simulink model "single_phase_afe_ideal"  (R2026a)
settings: Solver=ode23tb  StopTime=simlength  FixedStep=tc  MaxStep=glb_time.tc
values from neighbouring files (symbols this model uses):
  afe_ctrl = ctrl_afe_setup(glb_time.ts_afe, grid_emu.omega_grid_nom)    [init_model_legacy.m]
  frequency_set = 300    [init_model_legacy.m]
  glb_time = timing_setup(fpwm_afe, trgo_afe, fpwm_inv, trgo_inv, fpwm_single_phase_inv, trgo_single_phase_inv, fpwm_dab, trgo_dab,      fpwm_psfbc, trgo_psfbc, fpwm_isop_rail, trgo_isop_rail, fpwm_cllc, trgo_cllc, t_measure, tc_factor, tc_decimation, delay_pwm, dead_time_afe,      dead_time_inv, dead_time_single_phase_inv, dead_time_dab, dead_time_psfbc, dead_time_isop_rail, dead_time_cllc)    [init_model_legacy.m]
  grid_emu = grid_three_phase_emulator('Dyn11', delta_star, grid_nominal_power, application_voltage, us1, us2, fgrid,                  eq_grid_inductance, eq_grid_resistance, eta, ucc, i1m, p_iron, n1, n2, core_area, core_length, mur,                  up_xi_pu_ref, up_eta_pu_ref, un_xi_pu_ref, un_eta_pu_ref)    [init_model_legacy.m]
  heatsink = liquid_cooled_plate_2kw_setup(weight, no_weight, cp_al, heat_capacity_hs, thermal_conductivity_al,      Rth_switch_HA, Rth_mosfet_HA, Rth_diode_HA, Tambient, DThs_init)    [init_model_legacy.m]
  kepsilon = 2    [init_model_legacy.m]
  omega_set = frequency_set*2*pi    (= 1884.95559215)    [init_model_legacy.m]
  single_phase_inverter_ctrl = ctrl_single_phase_inverter_setup(glb_time.ts_inv, pres_ctrl.omega_set,      dqvector_pi.kp_inv, dqvector_pi.ki_inv, pres_ctrl.kp_rpi, pres_ctrl.ki_rpi, pres_ctrl.delta_rpi)    [init_model_legacy.m]
  Tambient = 40    [init_model_legacy.m]
  time_step_ref_1 = 0.025    [init_model_legacy.m]
  time_step_ref_2 = 0.5    [init_model_legacy.m]
  time_step_ref_3 = 1    [init_model_legacy.m]
  Vdc_nom = 400*1.35    (= 540)    [power_losses_calculation.m]
undefined symbols (not defined in the file or in its folder): delta_fht1, hwdata, igbt, Ld_fht1, magnitude, omega_fht1, ts_inv, Vac_FS, Xbez
libraries: fl_lib x116, nesl_utility x65, phase_shift_filter_ccaller x5, dq_vector_pi x4, igbt_simple_2th_lib x4, linear_double_integrator_observer_ccaller x3, lithium_ion_battery x1, dclink_for_two_levels x1, three_phase_voltage_with_frt_emulator x1, simulink x1, cstblocks_lti x1, single_phase_pwm_modulator x1
(part 5 of 6)

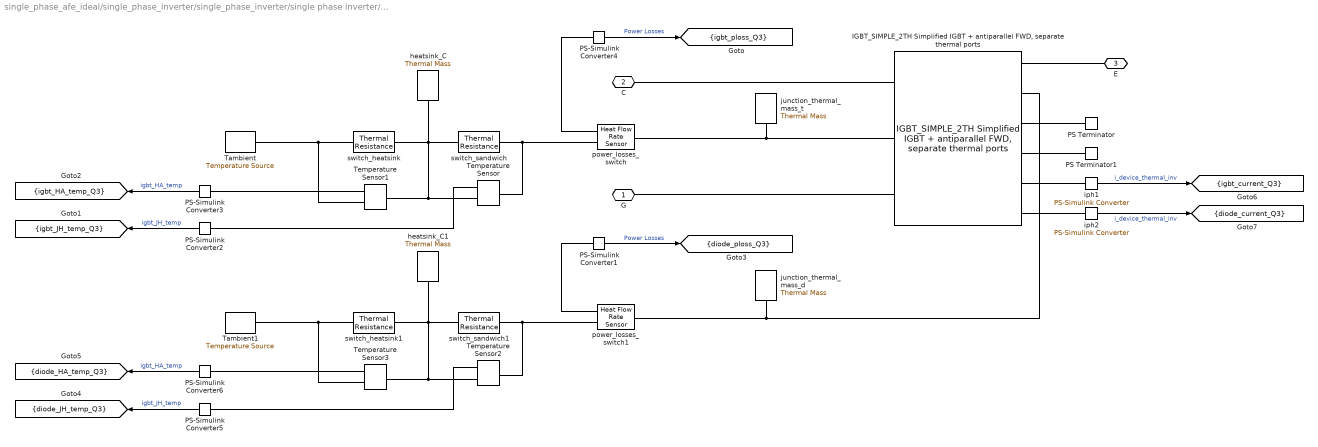
== system single_phase_afe_ideal/single_phase_inverter/single_phase_inverter/single phase inverter/three_phase_inverter_with_igbt_simple_2th/full_bridge_with_igbt_simple_2th/igbt_simple_3/IGBT_simple ==
  "IGBT_SIMPLE_2TH Simplified IGBT + antiparallel FWD, separate thermal ports" : igbt_simple_2th_lib/IGBT_SIMPLE_2TH Simplified IGBT + antiparallel FWD, separate thermal ports  Vce_sat=vce_sat_m V  Vf=v_gamma_m V  Vth=Vth_gate_m V  Vhyst=Vth_gate_hyst_m V  Eon_ref=Eon_m mJ  Eoff_ref=Eoff_m mJ  Err_ref=Err_m mJ  Ic_ref=Ic_ref_m A  Vdc_ref=Vdc_ref_m V  V_rr_th=Vblock_Errf_m V  Ron=rce_on_m mOhm  Rd=rd_on_m mOhm  Goff=Gce_off_m 1/Ohm  tau_s=time_constant_edge_m us  tau_p=time_constant_ploss_m us  i_specify=off  i_priority=None  i=0 A  i_nominal_specify=off  i_nominal_value=1  i_nominal_unit=A  v_specify=off  v_priority=None  v=0 V  v_nominal_specify=off  v_nominal_value=1  v_nominal_unit=V  i_t_specify=off  i_t_priority=None  i_t=0 A  i_t_nominal_specify=off  i_t_nominal_value=1  i_t_nominal_unit=A  i_d_specify=off  i_d_priority=None  i_d=0 A  i_d_nominal_specify=off  i_d_nominal_value=1  i_d_nominal_unit=A  i_h_specify=off  i_h_priority=None  i_h=0 A  i_h_nominal_specify=off  i_h_nominal_value=1  i_h_nominal_unit=A  i_dh_specify=off  i_dh_priority=None  i_dh=0 A  i_dh_nominal_specify=off  i_dh_nominal_value=1  i_dh_nominal_unit=A  v_h_specify=off  v_h_priority=None  v_h=0 V  v_h_nominal_specify=off  v_h_nominal_value=1  v_h_nominal_unit=V  E_lpt_specify=off  E_lpt_priority=None  E_lpt=0 J  E_lpt_nominal_specify=off  E_lpt_nominal_value=1  E_lpt_nominal_unit=J  E_lpd_specify=off  E_lpd_priority=None  E_lpd=0 J  E_lpd_nominal_specify=off  E_lpd_nominal_value=1  E_lpd_nominal_unit=J  Qt_specify=off  Qt_priority=None  Qt=0 W  Qt_nominal_specify=off  Qt_nominal_value=1  Qt_nominal_unit=W  Qd_specify=off  Qd_priority=None  Qd=0 W  Qd_nominal_specify=off  Qd_nominal_value=1  Qd_nominal_unit=W  E_t_specify=off  E_t_priority=None  E_t=0 J  E_d_specify=off  E_d_priority=None  E_d=0 J
  PS Terminator : fl_lib/Physical Signals/Sinks/PS Terminator
  PS Terminator1 : fl_lib/Physical Signals/Sinks/PS Terminator
  PS-Simulink Converter1 : nesl_utility/PS-Simulink Converter  PhysicalDomain=network_engine_domain  SubClassName=ps_output  LeftPortType=input  RightPortType=output  PseudoPeriodic=off  Frequencies=[]  VectorFormat=1-D array  Unit=J/s  AffineConversion=off
  PS-Simulink Converter{2..3,5..6} (4 alike) : nesl_utility/PS-Simulink Converter  PhysicalDomain=network_engine_domain  SubClassName=ps_output  LeftPortType=input  RightPortType=output  PseudoPeriodic=off  Frequencies=[]  VectorFormat=1-D array  Unit=degC  AffineConversion=off
  PS-Simulink Converter4 : nesl_utility/PS-Simulink Converter  PhysicalDomain=network_engine_domain  SubClassName=ps_output  LeftPortType=input  RightPortType=output  PseudoPeriodic=off  Frequencies=[]  VectorFormat=1-D array  Unit=J/s  AffineConversion=off
  Tambient : fl_lib/Thermal/Thermal Sources/Temperature Source  temperature=Tambient_m degC
  Tambient1 : fl_lib/Thermal/Thermal Sources/Temperature Source  temperature=Tambient_m degC
  Temperature Sensor{,1..3} (4 alike) : fl_lib/Thermal/Thermal Sensors/Temperature Sensor  temperature_measure=foundation.enum.MeasurementReference.difference
  heatsink_C : fl_lib/Thermal/Thermal Elements/Thermal Mass  mass_type=foundation.enum.constant_variable.constant  mass=mass_heatsink_m kg  sp_heat=specific_heat_m J/(K*kg)  mass_min=1e-6 kg  num_ports=foundation.enum.numPorts2.one  m_specify=off  m_priority=High  m=1 kg  m_nominal_specify=off  m_nominal_value=1  m_nominal_unit=kg  T_specify=on  T_priority=High  T=Tambient_m degC  T_nominal_specify=off  T_nominal_value=1  T_nominal_unit=K  Q_specify=off  Q_priority=High  Q=0 W  Q_nominal_specify=off  Q_nominal_value=1  Q_nominal_unit=W
  heatsink_C1 : fl_lib/Thermal/Thermal Elements/Thermal Mass  mass_type=foundation.enum.constant_variable.constant  mass=mass_heatsink_m kg  sp_heat=specific_heat_m J/(K*kg)  mass_min=1e-6 kg  num_ports=foundation.enum.numPorts2.one  m_specify=off  m_priority=High  m=1 kg  m_nominal_specify=off  m_nominal_value=1  m_nominal_unit=kg  T_specify=on  T_priority=High  T=Tambient_m degC  T_nominal_specify=off  T_nominal_value=1  T_nominal_unit=K  Q_specify=off  Q_priority=High  Q=0 W  Q_nominal_specify=off  Q_nominal_value=1  Q_nominal_unit=W
  iph1 : nesl_utility/PS-Simulink Converter  PhysicalDomain=network_engine_domain  SubClassName=ps_output  LeftPortType=input  RightPortType=output  PseudoPeriodic=off  Frequencies=[]  VectorFormat=1-D array  Unit=A  AffineConversion=off
  iph2 : nesl_utility/PS-Simulink Converter  PhysicalDomain=network_engine_domain  SubClassName=ps_output  LeftPortType=input  RightPortType=output  PseudoPeriodic=off  Frequencies=[]  VectorFormat=1-D array  Unit=A  AffineConversion=off
  junction_thermal_mass_d : fl_lib/Thermal/Thermal Elements/Thermal Mass  mass_type=foundation.enum.constant_variable.constant  mass=JunctionTermalMass_m/specific_heat_m kg  sp_heat=specific_heat_m J/(K*kg)  mass_min=1e-6 kg  num_ports=foundation.enum.numPorts2.one  m_specify=off  m_priority=High  m=1 kg  m_nominal_specify=off  m_nominal_value=1  m_nominal_unit=kg  T_specify=on  T_priority=High  T=Tambient_m degC  T_nominal_specify=off  T_nominal_value=1  T_nominal_unit=K  Q_specify=off  Q_priority=High  Q=0 W  Q_nominal_specify=off  Q_nominal_value=1  Q_nominal_unit=W
  junction_thermal_mass_t : fl_lib/Thermal/Thermal Elements/Thermal Mass  mass_type=foundation.enum.constant_variable.constant  mass=JunctionTermalMass_m/specific_heat_m kg  sp_heat=specific_heat_m J/(K*kg)  mass_min=1e-6 kg  num_ports=foundation.enum.numPorts2.one  m_specify=off  m_priority=High  m=1 kg  m_nominal_specify=off  m_nominal_value=1  m_nominal_unit=kg  T_specify=on  T_priority=High  T=Tambient_m degC  T_nominal_specify=off  T_nominal_value=1  T_nominal_unit=K  Q_specify=off  Q_priority=High  Q=0 W  Q_nominal_specify=off  Q_nominal_value=1  Q_nominal_unit=W
  power_losses_switch : fl_lib/Thermal/Thermal Sensors/Heat Flow Rate Sensor
  power_losses_switch1 : fl_lib/Thermal/Thermal Sensors/Heat Flow Rate Sensor
  switch_heatsink : fl_lib/Thermal/Thermal Elements/Thermal Resistance  resistance=rth_switch_HA_m K/W  T_specify=off  T_priority=High  T=0 deltadegC  T_nominal_specify=off  T_nominal_value=1  T_nominal_unit=K  Q_specify=off  Q_priority=None  Q=0 W  Q_nominal_specify=off  Q_nominal_value=1  Q_nominal_unit=W
  switch_heatsink1 : fl_lib/Thermal/Thermal Elements/Thermal Resistance  resistance=rth_diode_HA_m K/W  T_specify=off  T_priority=High  T=0 deltadegC  T_nominal_specify=off  T_nominal_value=1  T_nominal_unit=K  Q_specify=off  Q_priority=None  Q=0 W  Q_nominal_specify=off  Q_nominal_value=1  Q_nominal_unit=W
  switch_sandwich : fl_lib/Thermal/Thermal Elements/Thermal Resistance  resistance=rth_switch_JH_m K/W  T_specify=off  T_priority=High  T=0 degC  T_nominal_specify=off  T_nominal_value=1  T_nominal_unit=K  Q_specify=off  Q_priority=None  Q=0 W  Q_nominal_specify=off  Q_nominal_value=1  Q_nominal_unit=W
  switch_sandwich1 : fl_lib/Thermal/Thermal Elements/Thermal Resistance  resistance=rth_diode_JH_m K/W  T_specify=off  T_priority=High  T=0 degC  T_nominal_specify=off  T_nominal_value=1  T_nominal_unit=K  Q_specify=off  Q_priority=None  Q=0 W  Q_nominal_specify=off  Q_nominal_value=1  Q_nominal_unit=W
  G : PMIOPort  Side=Left
  C : PMIOPort  Port=2  Side=Left
  E : PMIOPort  Port=3  Side=Right
  tag scope: diode_HA_temp_Q3=scoped, diode_JH_temp_Q3=scoped, diode_current_Q3=scoped, diode_ploss_Q3=scoped, igbt_HA_temp_Q3=scoped, igbt_JH_temp_Q3=scoped, igbt_current_Q3=scoped, igbt_ploss_Q3=scoped
  wires:
  PS-Simulink Converter3/1 -> [igbt_HA_temp_Q3]  "igbt_HA_temp"
  PS-Simulink Converter4/1 -> [igbt_ploss_Q3]  "Power Losses"
  PS-Simulink Converter2/1 -> [igbt_JH_temp_Q3]  "igbt_JH_temp"
  PS-Simulink Converter1/1 -> [diode_ploss_Q3]  "Power Losses"
  PS-Simulink Converter5/1 -> [diode_JH_temp_Q3]  "igbt_JH_temp"
  PS-Simulink Converter6/1 -> [diode_HA_temp_Q3]  "igbt_HA_temp"
  iph1/1 -> [igbt_current_Q3]  "i_device_thermal_inv"
  iph2/1 -> [diode_current_Q3]  "i_device_thermal_inv"
  connections:
  Temperature Sensor/RConn2 -- PS-Simulink Converter2/LConn1
  "IGBT_SIMPLE_2TH Simplified IGBT + antiparallel FWD, separate thermal ports"/LConn2 -- junction_thermal_mass_t/LConn1 -- power_losses_switch/LConn1
  Temperature Sensor1/RConn2 -- PS-Simulink Converter3/LConn1
  switch_heatsink/LConn1 -- heatsink_C/LConn1 -- switch_sandwich/RConn1 -- Temperature Sensor1/LConn1 -- Temperature Sensor/RConn1
  switch_heatsink/RConn1 -- Tambient/LConn1 -- Temperature Sensor1/RConn1
  switch_sandwich/LConn1 -- power_losses_switch/RConn2 -- Temperature Sensor/LConn1
  "IGBT_SIMPLE_2TH Simplified IGBT + antiparallel FWD, separate thermal ports"/RConn1 -- E/RConn1
  "IGBT_SIMPLE_2TH Simplified IGBT + antiparallel FWD, separate thermal ports"/LConn1 -- C/RConn1
  "IGBT_SIMPLE_2TH Simplified IGBT + antiparallel FWD, separate thermal ports"/LConn3 -- G/RConn1
  Temperature Sensor2/RConn1 -- Temperature Sensor3/LConn1 -- heatsink_C1/LConn1 -- switch_heatsink1/LConn1 -- switch_sandwich1/RConn1
  Tambient1/LConn1 -- switch_heatsink1/RConn1 -- Temperature Sensor3/RConn1
  power_losses_switch1/RConn2 -- switch_sandwich1/LConn1 -- Temperature Sensor2/LConn1
  Temperature Sensor3/RConn2 -- PS-Simulink Converter6/LConn1
  Temperature Sensor2/RConn2 -- PS-Simulink Converter5/LConn1
  power_losses_switch1/LConn1 -- junction_thermal_mass_d/LConn1 -- "IGBT_SIMPLE_2TH Simplified IGBT + antiparallel FWD, separate thermal ports"/RConn2
  iph1/LConn1 -- "IGBT_SIMPLE_2TH Simplified IGBT + antiparallel FWD, separate thermal ports"/RConn5
  iph2/LConn1 -- "IGBT_SIMPLE_2TH Simplified IGBT + antiparallel FWD, separate thermal ports"/RConn6
  "IGBT_SIMPLE_2TH Simplified IGBT + antiparallel FWD, separate thermal ports"/RConn3 -- PS Terminator/LConn1
  "IGBT_SIMPLE_2TH Simplified IGBT + antiparallel FWD, separate thermal ports"/RConn4 -- PS Terminator1/LConn1
  PS-Simulink Converter1/LConn1 -- power_losses_switch1/RConn1
  PS-Simulink Converter4/LConn1 -- power_losses_switch/RConn1

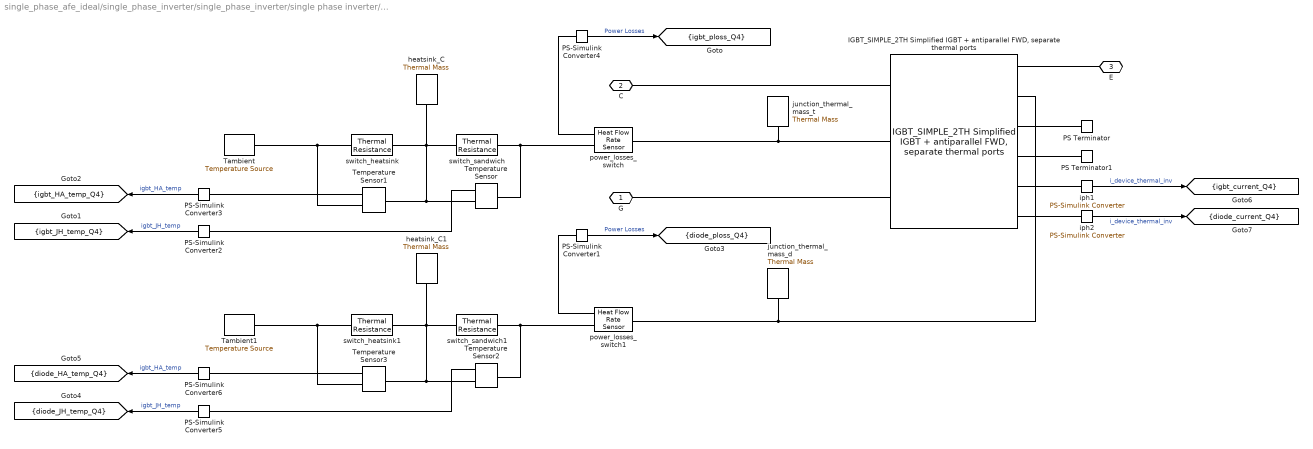
== system single_phase_afe_ideal/single_phase_inverter/single_phase_inverter/single phase inverter/three_phase_inverter_with_igbt_simple_2th/full_bridge_with_igbt_simple_2th/igbt_simple_4/IGBT_simple ==
  "IGBT_SIMPLE_2TH Simplified IGBT + antiparallel FWD, separate thermal ports" : igbt_simple_2th_lib/IGBT_SIMPLE_2TH Simplified IGBT + antiparallel FWD, separate thermal ports  Vce_sat=vce_sat_m V  Vf=v_gamma_m V  Vth=Vth_gate_m V  Vhyst=Vth_gate_hyst_m V  Eon_ref=Eon_m mJ  Eoff_ref=Eoff_m mJ  Err_ref=Err_m mJ  Ic_ref=Ic_ref_m A  Vdc_ref=Vdc_ref_m V  V_rr_th=Vblock_Errf_m V  Ron=rce_on_m mOhm  Rd=rd_on_m mOhm  Goff=Gce_off_m 1/Ohm  tau_s=time_constant_edge_m us  tau_p=time_constant_ploss_m us  i_specify=off  i_priority=None  i=0 A  i_nominal_specify=off  i_nominal_value=1  i_nominal_unit=A  v_specify=off  v_priority=None  v=0 V  v_nominal_specify=off  v_nominal_value=1  v_nominal_unit=V  i_t_specify=off  i_t_priority=None  i_t=0 A  i_t_nominal_specify=off  i_t_nominal_value=1  i_t_nominal_unit=A  i_d_specify=off  i_d_priority=None  i_d=0 A  i_d_nominal_specify=off  i_d_nominal_value=1  i_d_nominal_unit=A  i_h_specify=off  i_h_priority=None  i_h=0 A  i_h_nominal_specify=off  i_h_nominal_value=1  i_h_nominal_unit=A  i_dh_specify=off  i_dh_priority=None  i_dh=0 A  i_dh_nominal_specify=off  i_dh_nominal_value=1  i_dh_nominal_unit=A  v_h_specify=off  v_h_priority=None  v_h=0 V  v_h_nominal_specify=off  v_h_nominal_value=1  v_h_nominal_unit=V  E_lpt_specify=off  E_lpt_priority=None  E_lpt=0 J  E_lpt_nominal_specify=off  E_lpt_nominal_value=1  E_lpt_nominal_unit=J  E_lpd_specify=off  E_lpd_priority=None  E_lpd=0 J  E_lpd_nominal_specify=off  E_lpd_nominal_value=1  E_lpd_nominal_unit=J  Qt_specify=off  Qt_priority=None  Qt=0 W  Qt_nominal_specify=off  Qt_nominal_value=1  Qt_nominal_unit=W  Qd_specify=off  Qd_priority=None  Qd=0 W  Qd_nominal_specify=off  Qd_nominal_value=1  Qd_nominal_unit=W  E_t_specify=off  E_t_priority=None  E_t=0 J  E_d_specify=off  E_d_priority=None  E_d=0 J
  PS Terminator : fl_lib/Physical Signals/Sinks/PS Terminator
  PS Terminator1 : fl_lib/Physical Signals/Sinks/PS Terminator
  PS-Simulink Converter1 : nesl_utility/PS-Simulink Converter  PhysicalDomain=network_engine_domain  SubClassName=ps_output  LeftPortType=input  RightPortType=output  PseudoPeriodic=off  Frequencies=[]  VectorFormat=1-D array  Unit=J/s  AffineConversion=off
  PS-Simulink Converter{2..3,5..6} (4 alike) : nesl_utility/PS-Simulink Converter  PhysicalDomain=network_engine_domain  SubClassName=ps_output  LeftPortType=input  RightPortType=output  PseudoPeriodic=off  Frequencies=[]  VectorFormat=1-D array  Unit=degC  AffineConversion=off
  PS-Simulink Converter4 : nesl_utility/PS-Simulink Converter  PhysicalDomain=network_engine_domain  SubClassName=ps_output  LeftPortType=input  RightPortType=output  PseudoPeriodic=off  Frequencies=[]  VectorFormat=1-D array  Unit=J/s  AffineConversion=off
  Tambient : fl_lib/Thermal/Thermal Sources/Temperature Source  temperature=Tambient_m degC
  Tambient1 : fl_lib/Thermal/Thermal Sources/Temperature Source  temperature=Tambient_m degC
  Temperature Sensor{,1..3} (4 alike) : fl_lib/Thermal/Thermal Sensors/Temperature Sensor  temperature_measure=foundation.enum.MeasurementReference.difference
  heatsink_C : fl_lib/Thermal/Thermal Elements/Thermal Mass  mass_type=foundation.enum.constant_variable.constant  mass=mass_heatsink_m kg  sp_heat=specific_heat_m J/(K*kg)  mass_min=1e-6 kg  num_ports=foundation.enum.numPorts2.one  m_specify=off  m_priority=High  m=1 kg  m_nominal_specify=off  m_nominal_value=1  m_nominal_unit=kg  T_specify=on  T_priority=High  T=Tambient_m degC  T_nominal_specify=off  T_nominal_value=1  T_nominal_unit=K  Q_specify=off  Q_priority=High  Q=0 W  Q_nominal_specify=off  Q_nominal_value=1  Q_nominal_unit=W
  heatsink_C1 : fl_lib/Thermal/Thermal Elements/Thermal Mass  mass_type=foundation.enum.constant_variable.constant  mass=mass_heatsink_m kg  sp_heat=specific_heat_m J/(K*kg)  mass_min=1e-6 kg  num_ports=foundation.enum.numPorts2.one  m_specify=off  m_priority=High  m=1 kg  m_nominal_specify=off  m_nominal_value=1  m_nominal_unit=kg  T_specify=on  T_priority=High  T=Tambient_m degC  T_nominal_specify=off  T_nominal_value=1  T_nominal_unit=K  Q_specify=off  Q_priority=High  Q=0 W  Q_nominal_specify=off  Q_nominal_value=1  Q_nominal_unit=W
  iph1 : nesl_utility/PS-Simulink Converter  PhysicalDomain=network_engine_domain  SubClassName=ps_output  LeftPortType=input  RightPortType=output  PseudoPeriodic=off  Frequencies=[]  VectorFormat=1-D array  Unit=A  AffineConversion=off
  iph2 : nesl_utility/PS-Simulink Converter  PhysicalDomain=network_engine_domain  SubClassName=ps_output  LeftPortType=input  RightPortType=output  PseudoPeriodic=off  Frequencies=[]  VectorFormat=1-D array  Unit=A  AffineConversion=off
  junction_thermal_mass_d : fl_lib/Thermal/Thermal Elements/Thermal Mass  mass_type=foundation.enum.constant_variable.constant  mass=JunctionTermalMass_m/specific_heat_m kg  sp_heat=specific_heat_m J/(K*kg)  mass_min=1e-6 kg  num_ports=foundation.enum.numPorts2.one  m_specify=off  m_priority=High  m=1 kg  m_nominal_specify=off  m_nominal_value=1  m_nominal_unit=kg  T_specify=on  T_priority=High  T=Tambient_m degC  T_nominal_specify=off  T_nominal_value=1  T_nominal_unit=K  Q_specify=off  Q_priority=High  Q=0 W  Q_nominal_specify=off  Q_nominal_value=1  Q_nominal_unit=W
  junction_thermal_mass_t : fl_lib/Thermal/Thermal Elements/Thermal Mass  mass_type=foundation.enum.constant_variable.constant  mass=JunctionTermalMass_m/specific_heat_m kg  sp_heat=specific_heat_m J/(K*kg)  mass_min=1e-6 kg  num_ports=foundation.enum.numPorts2.one  m_specify=off  m_priority=High  m=1 kg  m_nominal_specify=off  m_nominal_value=1  m_nominal_unit=kg  T_specify=on  T_priority=High  T=Tambient_m degC  T_nominal_specify=off  T_nominal_value=1  T_nominal_unit=K  Q_specify=off  Q_priority=High  Q=0 W  Q_nominal_specify=off  Q_nominal_value=1  Q_nominal_unit=W
  power_losses_switch : fl_lib/Thermal/Thermal Sensors/Heat Flow Rate Sensor
  power_losses_switch1 : fl_lib/Thermal/Thermal Sensors/Heat Flow Rate Sensor
  switch_heatsink : fl_lib/Thermal/Thermal Elements/Thermal Resistance  resistance=rth_switch_HA_m K/W  T_specify=off  T_priority=High  T=0 deltadegC  T_nominal_specify=off  T_nominal_value=1  T_nominal_unit=K  Q_specify=off  Q_priority=None  Q=0 W  Q_nominal_specify=off  Q_nominal_value=1  Q_nominal_unit=W
  switch_heatsink1 : fl_lib/Thermal/Thermal Elements/Thermal Resistance  resistance=rth_diode_HA_m K/W  T_specify=off  T_priority=High  T=0 deltadegC  T_nominal_specify=off  T_nominal_value=1  T_nominal_unit=K  Q_specify=off  Q_priority=None  Q=0 W  Q_nominal_specify=off  Q_nominal_value=1  Q_nominal_unit=W
  switch_sandwich : fl_lib/Thermal/Thermal Elements/Thermal Resistance  resistance=rth_switch_JH_m K/W  T_specify=off  T_priority=High  T=0 degC  T_nominal_specify=off  T_nominal_value=1  T_nominal_unit=K  Q_specify=off  Q_priority=None  Q=0 W  Q_nominal_specify=off  Q_nominal_value=1  Q_nominal_unit=W
  switch_sandwich1 : fl_lib/Thermal/Thermal Elements/Thermal Resistance  resistance=rth_diode_JH_m K/W  T_specify=off  T_priority=High  T=0 degC  T_nominal_specify=off  T_nominal_value=1  T_nominal_unit=K  Q_specify=off  Q_priority=None  Q=0 W  Q_nominal_specify=off  Q_nominal_value=1  Q_nominal_unit=W
  G : PMIOPort  Side=Left
  C : PMIOPort  Port=2  Side=Left
  E : PMIOPort  Port=3  Side=Right
  tag scope: diode_HA_temp_Q4=scoped, diode_JH_temp_Q4=scoped, diode_current_Q4=scoped, diode_ploss_Q4=scoped, igbt_HA_temp_Q4=scoped, igbt_JH_temp_Q4=scoped, igbt_current_Q4=scoped, igbt_ploss_Q4=scoped
  wires:
  iph2/1 -> [diode_current_Q4]  "i_device_thermal_inv"
  iph1/1 -> [igbt_current_Q4]  "i_device_thermal_inv"
  PS-Simulink Converter6/1 -> [diode_HA_temp_Q4]  "igbt_HA_temp"
  PS-Simulink Converter5/1 -> [diode_JH_temp_Q4]  "igbt_JH_temp"
  PS-Simulink Converter1/1 -> [diode_ploss_Q4]  "Power Losses"
  PS-Simulink Converter2/1 -> [igbt_JH_temp_Q4]  "igbt_JH_temp"
  PS-Simulink Converter4/1 -> [igbt_ploss_Q4]  "Power Losses"
  PS-Simulink Converter3/1 -> [igbt_HA_temp_Q4]  "igbt_HA_temp"
  connections:
  iph2/LConn1 -- "IGBT_SIMPLE_2TH Simplified IGBT + antiparallel FWD, separate thermal ports"/RConn6
  iph1/LConn1 -- "IGBT_SIMPLE_2TH Simplified IGBT + antiparallel FWD, separate thermal ports"/RConn5
  power_losses_switch1/LConn1 -- junction_thermal_mass_d/LConn1 -- "IGBT_SIMPLE_2TH Simplified IGBT + antiparallel FWD, separate thermal ports"/RConn2
  Temperature Sensor2/RConn2 -- PS-Simulink Converter5/LConn1
  Temperature Sensor3/RConn2 -- PS-Simulink Converter6/LConn1
  Temperature Sensor2/LConn1 -- switch_sandwich1/LConn1 -- power_losses_switch1/RConn2
  Temperature Sensor3/RConn1 -- switch_heatsink1/RConn1 -- Tambient1/LConn1
  switch_sandwich1/RConn1 -- switch_heatsink1/LConn1 -- heatsink_C1/LConn1 -- Temperature Sensor3/LConn1 -- Temperature Sensor2/RConn1
  "IGBT_SIMPLE_2TH Simplified IGBT + antiparallel FWD, separate thermal ports"/LConn3 -- G/RConn1
  "IGBT_SIMPLE_2TH Simplified IGBT + antiparallel FWD, separate thermal ports"/LConn1 -- C/RConn1
  "IGBT_SIMPLE_2TH Simplified IGBT + antiparallel FWD, separate thermal ports"/RConn1 -- E/RConn1
  Temperature Sensor/LConn1 -- power_losses_switch/RConn2 -- switch_sandwich/LConn1
  Temperature Sensor1/RConn1 -- Tambient/LConn1 -- switch_heatsink/RConn1
  Temperature Sensor/RConn1 -- Temperature Sensor1/LConn1 -- switch_sandwich/RConn1 -- heatsink_C/LConn1 -- switch_heatsink/LConn1
  Temperature Sensor1/RConn2 -- PS-Simulink Converter3/LConn1
  "IGBT_SIMPLE_2TH Simplified IGBT + antiparallel FWD, separate thermal ports"/LConn2 -- junction_thermal_mass_t/LConn1 -- power_losses_switch/LConn1
  Temperature Sensor/RConn2 -- PS-Simulink Converter2/LConn1
  PS Terminator/LConn1 -- "IGBT_SIMPLE_2TH Simplified IGBT + antiparallel FWD, separate thermal ports"/RConn3
  "IGBT_SIMPLE_2TH Simplified IGBT + antiparallel FWD, separate thermal ports"/RConn4 -- PS Terminator1/LConn1
  PS-Simulink Converter4/LConn1 -- power_losses_switch/RConn1
  PS-Simulink Converter1/LConn1 -- power_losses_switch1/RConn1

== system single_phase_afe_ideal/single_phase_inverter/single phase inverter control/single_phase_inverter_ctrl/phase generator/FHT-PLL/pll_stageA/filter_and_transformation/FHTalpha ==
  u : Inport
  Bus Selector : BusSelector  OutputSignals=output_pu_hat,output_pu_hat_dot
  C Caller : CCaller  FunctionName=first_harmonic_tracker_process_simulink  PortSpecificationStruct="%)30     .    B \\   8    (     @         %    \"     D    !     0         %  0 \"0    $    _    07)G3F%M90  4&]R=$YA;64 4V-O<&4     26YD97@     5'EP90      4VEZ90      27-';&]B86P   X    P    !@    @    $          4    (     0    ,    !         !   P!O=70 #@   #     &    \"     0         !0    @    !     P    $         $  # &]U=  .    .     8    (    !          %    \"     $    &     0         0  ...(+4988 chars)"
  Constant : Constant  Value=glb_time.ts_afe
  Constant1 : Constant  Value=0
  Constant4 : Constant  Value=afe_ctrl.fht_grid.omega_fht
  Constant5 : Constant  Value=afe_ctrl.fht_grid.delta_fht
  Constant6 : Constant  Value=afe_ctrl.fht_grid.Ld_fht(1)
  Constant7 : Constant  Value=afe_ctrl.fht_grid.Ld_fht(2)
  Data Type Conversion{1..2,6..9} (6 alike) : DataTypeConversion  OutDataTypeStr=single  SaturateOnIntegerOverflow=off  RndMeth=Floor
  Data Type Conversion10 : DataTypeConversion  OutDataTypeStr=double  SaturateOnIntegerOverflow=off  RndMeth=Floor
  Data Type Conversion3 : DataTypeConversion  OutDataTypeStr=uint8  SaturateOnIntegerOverflow=off  RndMeth=Floor
  Data Type Conversion4 : DataTypeConversion  OutDataTypeStr=double  SaturateOnIntegerOverflow=off  RndMeth=Floor
  Data Type Conversion5 : DataTypeConversion  OutDataTypeStr=uint8  SaturateOnIntegerOverflow=off  RndMeth=Floor
  Gain : Gain  Gain=1/afe_ctrl.fht_grid.omega_fht
  Step : Step  Time=0.0125  InitialValue=1  FinalValue=0
  ud_hat : Outport
  uq_hat : Outport  Port=2
  wires:
  Data Type Conversion9/1 -> C Caller/7
  Data Type Conversion8/1 -> C Caller/6
  Data Type Conversion7/1 -> C Caller/5
  Data Type Conversion6/1 -> C Caller/4
  Data Type Conversion5/1 -> C Caller/8
  Constant5/1 -> Data Type Conversion7/1
  Constant7/1 -> Data Type Conversion9/1
  Constant6/1 -> Data Type Conversion8/1
  Constant4/1 -> Data Type Conversion6/1
  Constant1/1 -> Data Type Conversion5/1
  Constant/1 -> Data Type Conversion1/1
  u/1 -> Data Type Conversion2/1
  Step/1 -> Data Type Conversion3/1
  Bus Selector/1 -> Data Type Conversion4/1  "<output_pu_hat>"
  C Caller/1 -> Bus Selector/1
  Data Type Conversion2/1 -> C Caller/2
  Data Type Conversion1/1 -> C Caller/3
  Data Type Conversion3/1 -> C Caller/1
  Data Type Conversion4/1 -> ud_hat/1
  Data Type Conversion10/1 -> Gain/1
  Bus Selector/2 -> Data Type Conversion10/1  "<output_pu_hat_dot>"
  Gain/1 -> uq_hat/1

== system single_phase_afe_ideal/single_phase_inverter/single phase inverter control/single_phase_inverter_ctrl/phase generator/FHT-PLL/pll_stageA/filter_and_transformation/FHTbeta ==
  u : Inport
  Bus Selector : BusSelector  OutputSignals=output_pu_hat,output_pu_hat_dot
  C Caller : CCaller  FunctionName=first_harmonic_tracker_process_simulink  PortSpecificationStruct="%)30     .    B \\   8    (     @         %    \"     D    !     0         %  0 \"0    $    _    07)G3F%M90  4&]R=$YA;64 4V-O<&4     26YD97@     5'EP90      4VEZ90      27-';&]B86P   X    P    !@    @    $          4    (     0    ,    !         !   P!O=70 #@   #     &    \"     0         !0    @    !     P    $         $  # &]U=  .    .     8    (    !          %    \"     $    &     0         0  ...(+4988 chars)"
  Constant : Constant  Value=glb_time.ts_afe
  Constant1 : Constant  Value=2
  Constant4 : Constant  Value=afe_ctrl.fht_grid.omega_fht
  Constant5 : Constant  Value=afe_ctrl.fht_grid.delta_fht
  Constant6 : Constant  Value=afe_ctrl.fht_grid.Ld_fht(1)
  Constant7 : Constant  Value=afe_ctrl.fht_grid.Ld_fht(2)
  Data Type Conversion{1..2,6..9} (6 alike) : DataTypeConversion  OutDataTypeStr=single  SaturateOnIntegerOverflow=off  RndMeth=Floor
  Data Type Conversion10 : DataTypeConversion  OutDataTypeStr=double  SaturateOnIntegerOverflow=off  RndMeth=Floor
  Data Type Conversion3 : DataTypeConversion  OutDataTypeStr=uint8  SaturateOnIntegerOverflow=off  RndMeth=Floor
  Data Type Conversion4 : DataTypeConversion  OutDataTypeStr=double  SaturateOnIntegerOverflow=off  RndMeth=Floor
  Data Type Conversion5 : DataTypeConversion  OutDataTypeStr=uint8  SaturateOnIntegerOverflow=off  RndMeth=Floor
  Gain : Gain  Gain=1/afe_ctrl.fht_grid.omega_fht
  Step : Step  Time=0.0125  InitialValue=1  FinalValue=0
  ud_hat : Outport
  uq_hat : Outport  Port=2
  wires:
  Gain/1 -> uq_hat/1
  Bus Selector/2 -> Data Type Conversion10/1  "<output_pu_hat_dot>"
  Data Type Conversion10/1 -> Gain/1
  Data Type Conversion4/1 -> ud_hat/1
  Data Type Conversion3/1 -> C Caller/1
  Data Type Conversion1/1 -> C Caller/3
  Data Type Conversion2/1 -> C Caller/2
  C Caller/1 -> Bus Selector/1
  Bus Selector/1 -> Data Type Conversion4/1  "<output_pu_hat>"
  Step/1 -> Data Type Conversion3/1
  u/1 -> Data Type Conversion2/1
  Constant/1 -> Data Type Conversion1/1
  Constant1/1 -> Data Type Conversion5/1
  Constant4/1 -> Data Type Conversion6/1
  Constant6/1 -> Data Type Conversion8/1
  Constant7/1 -> Data Type Conversion9/1
  Constant5/1 -> Data Type Conversion7/1
  Data Type Conversion5/1 -> C Caller/8
  Data Type Conversion6/1 -> C Caller/4
  Data Type Conversion7/1 -> C Caller/5
  Data Type Conversion8/1 -> C Caller/6
  Data Type Conversion9/1 -> C Caller/7

== system single_phase_afe_ideal/single_phase_inverter/single phase inverter control/single_phase_inverter_ctrl/single_phase_current_control/dqpi_current_controller/i2alphabeta/sogi/integrator_1 ==
  in : Inport
  Sum : Sum  Inputs=|++
  sample_time : Gain  Gain=glb_time.ts_inv
  unit_delay_1 : UnitDelay  SampleTime=-1
  out : Outport
  wires:
  in/1 -> sample_time/1
  sample_time/1 -> Sum/1
  Sum/1 -> unit_delay_1/1, out/1
  unit_delay_1/1 -> Sum/2

== system single_phase_afe_ideal/single_phase_inverter/single phase inverter control/single_phase_inverter_ctrl/single_phase_current_control/dqpi_current_controller/i2alphabeta/sogi/integrator_2 ==
  in : Inport
  Sum : Sum  Inputs=|++
  sample_time : Gain  Gain=glb_time.ts_inv
  unit_delay_1 : UnitDelay  SampleTime=-1
  out : Outport
  wires:
  sample_time/1 -> Sum/1
  in/1 -> sample_time/1
  Sum/1 -> out/1, unit_delay_1/1
  unit_delay_1/1 -> Sum/2

== system single_phase_afe_ideal/single_phase_inverter/single phase inverter control/single_phase_inverter_ctrl/single_phase_current_control/dqpi_current_controller/i2alphabeta/sogi_ccaller/Reset ==
  Step : Step  Time=0.025  InitialValue=1  FinalValue=0
  en : Outport
  wires:
  Step/1 -> en/1

== matlab function single_phase_afe_ideal/single_phase_inverter/single phase inverter control/single_phase_inverter_ctrl/phase generator/FHT-PLL/pll_stageB/bounder1 ==
  data: u input; y output
function y = bounder(u)
    y = -pi + mod(u+3*pi,2*pi);
end

== matlab function single_phase_afe_ideal/single_phase_inverter/single phase inverter control/single_phase_inverter_ctrl/phase generator/FHT-PLL/pll_stageB/double_integrator_observer/bounder1 ==
  data: u input; y output
function y = bounder(u)
    
    y = -pi + mod(u+3*pi,2*pi);
    
end

== matlab function single_phase_afe_ideal/power meter iec mfunc/three_phase_power_meter_iec ==
  data: phase input; m output Bus: PowerMeterIecBus; u_abc input; i_abc input; omega input; ts input; enable_time input
function m = three_phase_power_meter_iec(phase, u_abc, i_abc, omega, ts, enable_time)
%#codegen
% THREE_PHASE_POWER_METER_IEC
% Equivalente in singolo blocco MATLAB Function del sottosistema Simulink
% "three_phase_power_meter_iec" (libreria power_meter_iec).
%
% INGRESSI
%   phase       : angolo del PLL [rad]      (scalare)
%   u_abc       : tensioni di fase [V]      (3x1)
%   i_abc       : correnti di linea [A]     (3x1)
%   omega       : pulsazione di rete [rad/s] (scalare)
%   ts          : passo di campionamento [s]  -> parametro di maschera
%   enable_time : istante di abilitazione [s] -> parametro di maschera
%
% USCITA
%   m : struct (bus) con i campi, nello stesso ordine del Bus Creator
%       originale: Q1p, Q1n, P1n, P1p, U1n, U1p,
%                  i_act_1n, i_react_1n, i_act_1p, i_react_1p
%
% CATENA DI ELABORAZIONE (identica all'originale)
%   1) proiezione di ogni fase su cos(phase) e sin(phase), guadagno 2
%   2) media mobile dinamica su finestra pari a mezzo periodo di rete
%      (Tw = pi/|omega|), con lunghezza frazionaria interpolata
%   3) componenti simmetriche di sequenza diretta e inversa (Fortescue)
%   4) potenze attiva e reattiva per sequenza, tensioni concatenate RMS,
%      correnti attiva e reattiva per sequenza
%
% NOTE
%   - Il blocco deve girare a passo fisso ts (gli Zero-Order Hold di
%     ingresso dell'originale sono impliciti nel sample time del blocco).
%   - ts ed enable_time possono essere dichiarati come dati di scope
%     "Parameter" nel Symbols pane del MATLAB Function block, cosi'
%     risolvono direttamente sui parametri di maschera e la firma
%     esterna resta a 4 ingressi come nel blocco originale.

% ------------------------------------------------------------------
% Costanti
% ------------------------------------------------------------------
% MAVGFLT_SIZE_MAX = 17500;   % lunghezza buffer circolare (come originale)
MAVGFLT_SIZE_MAX = 2048;   % lunghezza buffer ridotto
NCH              = 12;      % canali filtrati: 6 per u_abc, 6 per i_abc

% Ordine canali:
%   1..3  ua_cos ub_cos uc_cos      7..9   ia_cos ib_cos ic_cos
%   4..6  ua_sin ub_sin uc_sin     10..12  ia_sin ib_sin ic_sin

% ------------------------------------------------------------------
% Stato persistente
% ------------------------------------------------------------------
persistent buf cb_index sample_count sum_short sum_long prev_input ...
           k_step period_held

if isempty(buf)
    buf          = zeros(NCH, MAVGFLT_SIZE_MAX);
    cb_index     = ones(NCH, 1);
    sample_count = ones(NCH, 1);
    sum_short    = zeros(NCH, 1);
    sum_long     = zeros(NCH, 1);
    prev_input   = zeros(NCH, 1);
    k_step       = 0;
    period_held  = 0;          % uscita iniziale dell'Enabled Subsystem
end

% ------------------------------------------------------------------
% Abilitazione (equivalente al blocco Step con Time = enable_time)
% ------------------------------------------------------------------
t_now  = k_step * ts;
k_step = k_step + 1;
enable = (t_now >= enable_time);

% ------------------------------------------------------------------
% Finestra di media: Enabled Subsystem 2*pi/w, alimentato da 2*|omega|.
% Quando |omega| = 0 l'Enabled Subsystem mantiene l'ultimo valore.
% ------------------------------------------------------------------
w2 = 2 * abs(omega);
if w2 > 0
    period_held = 2*pi / w2;   % = pi/|omega|, mezzo periodo di rete
end
period = period_held;

% ------------------------------------------------------------------
% Proiezione sin/cos, guadagno 2
% ------------------------------------------------------------------
c = cos(phase);
s = sin(phase);

x = zeros(NCH, 1);
x(1)  = 2 * u_abc(1) * c;   x(2)  = 2 * u_abc(2) * c;   x(3)  = 2 * u_abc(3) * c;
x(4)  = 2 * u_abc(1) * s;   x(5)  = 2 * u_abc(2) * s;   x(6)  = 2 * u_abc(3) * s;
x(7)  = 2 * i_abc(1) * c;   x(8)  = 2 * i_abc(2) * c;   x(9)  = 2 * i_abc(3) * c;
x(10) = 2 * i_abc(1) * s;   x(11) = 2 * i_abc(2) * s;   x(12) = 2 * i_abc(3) * s;

% ------------------------------------------------------------------
% Banco di 12 filtri a media mobile dinamica (dmavgflt_process)
% ------------------------------------------------------------------
y = zeros(NCH, 1);

if enable && period > 0

    desired = period / ts;
    if desired > (MAVGFLT_SIZE_MAX - 1)
        desired = MAVGFLT_SIZE_MAX - 1;
    end

    n_samples = floor(desired + 1);          % campioni che coprono il periodo
    frac      = desired + 1 - n_samples;     % parte frazionaria
    if n_samples < 1
        n_samples = 1;
    end

    for ch = 1:NCH

        ci = cb_index(ch);
        sc = sample_count(ch);

        if n_samples > sc
            % finestra in crescita: aggiungi campioni
            sum_short(ch) = sum_short(ch) + prev_input(ch);
            sum_long(ch)  = sum_long(ch)  + x(ch);
            sc = sc + 1;

        elseif n_samples < sc
            % finestra in contrazione: rimuovi i due campioni piu' vecchi
            i1 = mod(ci - 1 - sc,       MAVGFLT_SIZE_MAX) + 1;
            i2 = mod(ci - 1 - (sc - 1), MAVGFLT_SIZE_MAX) + 1;
            old_sum = buf(ch, i1) + buf(ch, i2);

            sum_short(ch) = sum_short(ch) + prev_input(ch) - old_sum;
            sum_long(ch)  = sum_long(ch)  + x(ch)          - old_sum;
            sc = sc - 1;

        else
            % finestra costante
            i1     = mod(ci - 1 - sc, MAVGFLT_SIZE_MAX) + 1;
            oldest = buf(ch, i1);

            sum_short(ch) = sum_short(ch) + prev_input(ch) - oldest;
            sum_long(ch)  = sum_long(ch)  + x(ch)          - oldest;
        end

        % aggiornamento buffer circolare
        buf(ch, ci)      = x(ch);
        cb_index(ch)     = mod(ci, MAVGFLT_SIZE_MAX) + 1;
        prev_input(ch)   = x(ch);
        sample_count(ch) = sc;

        % uscita: interpolazione lineare fra finestra corta e lunga
        if sc > 1
            avg_short = sum_short(ch) / (sc - 1);
        else
            avg_short = 0;
        end
        avg_long = sum_long(ch) / sc;

        y(ch) = avg_short * (1 - frac) + avg_long * frac;
    end
end
% se enable = false oppure period <= 0: y resta 0 e lo stato non evolve
% (comportamento identico all'originale)

ua_cos = y(1);  ub_cos = y(2);  uc_cos = y(3);
ua_sin = y(4);  ub_sin = y(5);  uc_sin = y(6);
ia_cos = y(7);  ib_cos = y(8);  ic_cos = y(9);
ia_sin = y(10); ib_sin = y(11); ic_sin = y(12);

% ------------------------------------------------------------------
% Componenti simmetriche (fasori con convenzione U = u_cos - j*u_sin)
% ------------------------------------------------------------------
sq3 = sqrt(3);

u1p_cos = (2*ua_cos - ub_cos - uc_cos - sq3*(uc_sin - ub_sin)) / 6;
u1p_sin = (2*ua_sin - ub_sin - uc_sin - sq3*(ub_cos - uc_cos)) / 6;
u1n_cos = (2*ua_cos - ub_cos - uc_cos - sq3*(ub_sin - uc_sin)) / 6;
u1n_sin = (2*ua_sin - ub_sin - uc_sin - sq3*(uc_cos - ub_cos)) / 6;

i1p_cos = (2*ia_cos - ib_cos - ic_cos - sq3*(ic_sin - ib_sin)) / 6;
i1p_sin = (2*ia_sin - ib_sin - ic_sin - sq3*(ib_cos - ic_cos)) / 6;
i1n_cos = (2*ia_cos - ib_cos - ic_cos - sq3*(ib_sin - ic_sin)) / 6;
i1n_sin = (2*ia_sin - ib_sin - ic_sin - sq3*(ic_cos - ib_cos)) / 6;

% ------------------------------------------------------------------
% Potenze per sequenza
% ------------------------------------------------------------------
P1p = 1.5 * (u1p_cos*i1p_cos + u1p_sin*i1p_sin);
Q1p = 1.5 * (u1p_cos*i1p_sin - u1p_sin*i1p_cos);
P1n = 1.5 * (u1n_cos*i1n_cos + u1n_sin*i1n_sin);
Q1n = 1.5 * (u1n_cos*i1n_sin - u1n_sin*i1n_cos);

% ------------------------------------------------------------------
% Tensioni concatenate RMS per sequenza: sqrt(3/2)*ampiezza di fase
% ------------------------------------------------------------------
U1p = sqrt(1.5 * (u1p_cos^2 + u1p_sin^2));
U1n = sqrt(1.5 * (u1n_cos^2 + u1n_sin^2));

% ------------------------------------------------------------------
% Correnti attiva e reattiva per sequenza (RMS di linea)
% La protezione contro la divisione per zero non era presente nello
% schema originale (i blocchi Divide restituivano Inf/NaN a U = 0).
% Portare U_MIN a 0 per replicare esattamente il comportamento vecchio.
% ------------------------------------------------------------------
U_MIN = 1e-9;

if U1p > U_MIN
    i_act_1p   = P1p / (sq3 * U1p);
    i_react_1p = Q1p / (sq3 * U1p);
else
    i_act_1p   = 0;
    i_react_1p = 0;
end

if U1n > U_MIN
    i_act_1n   = P1n / (sq3 * U1n);
    i_react_1n = Q1n / (sq3 * U1n);
else
    i_act_1n   = 0;
    i_react_1n = 0;
end

% ------------------------------------------------------------------
% Bus di uscita (stesso ordine dei campi dell'originale)
% ------------------------------------------------------------------
m.Q1p        = Q1p;
m.Q1n        = Q1n;
m.P1n        = P1n;
m.P1p        = P1p;
m.U1n        = U1n;
m.U1p        = U1p;
m.i_act_1n   = i_act_1n;
m.i_react_1n = i_react_1n;
m.i_act_1p   = i_act_1p;
m.i_react_1p = i_react_1p;

end

== matlab function single_phase_afe_ideal/single_phase_inverter/single phase inverter control/single_phase_inverter_ctrl/dclink_ripple_compensation_dq/dq2alphabeta/MATLAB Function ==
  data: d input; alpha output; q input; phase input; beta output
function [alpha, beta] = dq2alphabeta(d, q, phase)

alpha = d*cos(phase) - q*sin(phase);
beta = d*sin(phase) + q*cos(phase);

== matlab function single_phase_afe_ideal/single_phase_inverter/single phase inverter control/single_phase_inverter_ctrl/dclink_ripple_compensation_rpi/alphabeta2dq/MATLAB Function ==
  data: alpha input; d output; beta input; phase input; q output
function [d, q] = alphabeta2dq(alpha, beta, phase)

d = alpha*cos(phase) + beta*sin(phase);
q = -alpha*sin(phase) + beta*cos(phase);
